simulink model "Prj2CDig_escalonado_gemeo_v2"  (R2026b)
settings: Solver=FixedStepDiscrete  StartTime=0  StopTime=StopTime  FixedStep=Ts
model workspace (MAT data in the model file):
  APlantCool = 0.758025026799
  APlantNom = [0.976809482048  0; 0  0.837999478908]
  BPlantCool = 0.0389974309185
  BPlantNom = [0.012391015895; 0.0114915598792]
  BetaCoolerSeno = 0.8
  CPlantCool = 0.00533973420046
  CPlantNom = [0.00104118199184 0.0230826408129]
  ConfirmacoesModo = 2
  FaseSeno = 2.9409972793
  KWVariavelParaPwm16 = 0
  Pwm16Max = 65535
  Pwm16Min = 0
  StopTime = 3600
  SubpassosGemeo = 6
  TaSim = 26.6
  Ts = 5.715
  TsSobre2 = 2.8575
  TsSubGemeo = 0.9525
  WBaseCooler = 3211
  WEntrarCooler = 2000
  WSairCooler = 1000
  YInicialGemeo = 27
  YInicialSim = 50
  cooler.y0 = 50
  cooler.u0 = 29668.6850394
  cooler.Nb = 2157.30127859
  cooler.Ki = 74.6363818008
  cooler.Kx = 9.0523214643
  cooler.Kq = 0.368257902254
  cooler.C = 0.00533973420046
  cooler.Cs = [1.21494479074 5.41983902077]
  cooler.Aod = [0.758025026799  0.0389974309185  0; 0  0.846686888484  5.41983902077; 0  -0.052237956106  0.846686888484]
  cooler.Bod = [0.0389974309185; 0; 0]
  cooler.Ld = [59.9192070008; -1100.25874176; -100.465858002]
  cooler.AdPlanta = 0.758025026799
  cooler.BdPlanta = 0.0389974309185
  cooler.CdPlanta = 0.00533973420046
  nominal.y0 = 50.50283
  nominal.u0 = 9688.13559322
  nominal.Nb = 1615.01542842
  nominal.Ki = 55.87486056
  nominal.Kx = [2.42292827 37.30035107]
  nominal.Kq = 0.45467056
  nominal.Cs = [1.30135744 5.41983902]
  nominal.GTermicoPwm16 = 455.85236927
  nominal.AdPlanta = [0.976809482048  0; 0  0.837999478908]
  nominal.BdPlanta = [0.012391015895; 0.0114915598792]
  nominal.CdPlanta = [0.00104118199184 0.0230826408129]
  nominal.Aod = [0.871488506271  -2.3349292179  0.012391015895  0; -0.0214603685254  0.362230610194  0.0114915598792  0; 0.547000658391  12.1268133919  0.846686888484  5.41983902077; 0.0988681165312  2.19187158404  -0.052237956106  0.846686888484]
  nominal.Bod = [0.012391015895; 0.0114915598792; 0; 0]
  nominal.Ld = [101.15520303; 20.6115440851; -525.365078033; -94.9575744738]
  nominal.Cod = [0.00104118199184 0.0230826408129 0 0]
  thetaGemeo = [0.00594308095276 0.00147339059286 0.0179875985617 0.0289186352165 1.00003134628e-05 0.0158089923599 4.45570940962e-05]
  vCenario = [5.715 26.6 3211 0.8 2.9409972793]
  vCool = [2.8575 50 29668.6850394 2157.30127859 74.6363818008 9.0523214643 0.368257902254 0.00533973420046 1.21494479074 5.41983902077]
  vNom = [2.8575 50.50283 9688.13559322 1615.01542842 55.87486056 2.42292827 37.30035107 0.45467056 1.30135744 5.41983902 455.85236927 0.976809482048 0.837999478908 0.012391015895 0.0114915598792]
  vPlanta = [50 50.50283 9688.13559322 50 29668.6850394 3211 0]
  vSupervisor = [2000 1000 2]
settings Model: Creator=Santana  LastModifiedBy=Santana

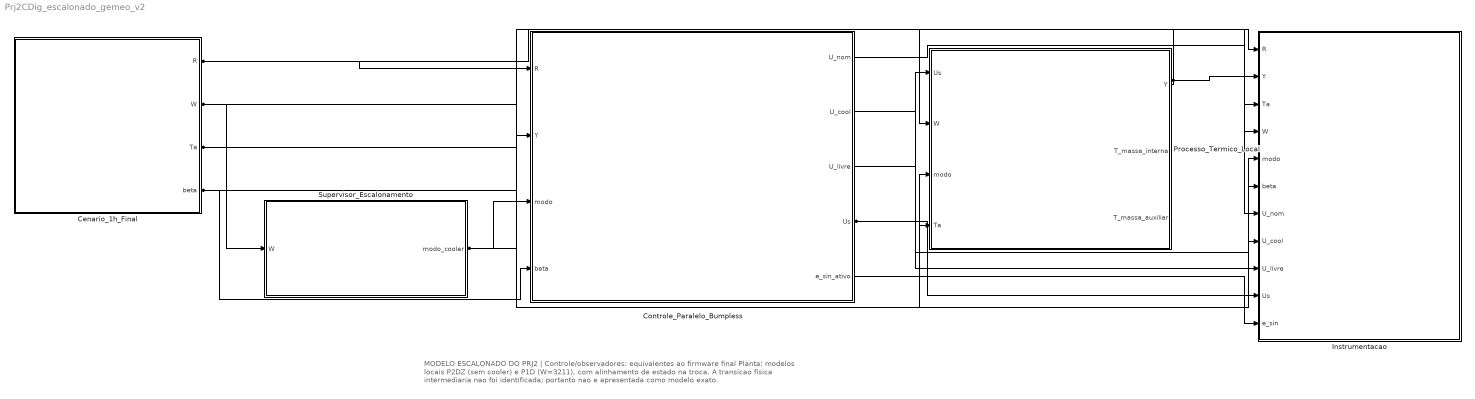
== system Prj2CDig_escalonado_gemeo_v2 ==
  note: MODELO ESCALONADO DO PRJ2  |  Controle/observadores: equivalentes ao firmware final
      | Planta: modelos locais P2DZ (sem cooler) e P1D (W=3211), com alinhamento de estado na troca.
      | A transicao fisica intermediaria nao foi identificada; portanto nao e apresentada como modelo exato.
  Cenario_1h_Final : Subsystem
  Controle_Paralelo_Bumpless : Subsystem
  Instrumentacao : Subsystem
  Processo_Termico_Local : Subsystem
  Supervisor_Escalonamento : Subsystem
  wires:
  Cenario_1h_Final/1(R) -> Controle_Paralelo_Bumpless/1(R), Instrumentacao/1(R)
  Cenario_1h_Final/2(W) -> Supervisor_Escalonamento/1(W), Processo_Termico_Local/2(W), Instrumentacao/4(W)
  Cenario_1h_Final/4(beta) -> Controle_Paralelo_Bumpless/4(beta), Instrumentacao/6(beta)
  Supervisor_Escalonamento/1(modo_cooler) -> Controle_Paralelo_Bumpless/3(modo), Processo_Termico_Local/3(modo), Instrumentacao/5(modo)
  Controle_Paralelo_Bumpless/4(Us) -> Processo_Termico_Local/1(Us), Instrumentacao/10(Us)
  Processo_Termico_Local/1(Y) -> Controle_Paralelo_Bumpless/2(Y), Instrumentacao/2(Y)
  Cenario_1h_Final/3(Ta) -> Instrumentacao/3(Ta), Processo_Termico_Local/4(Ta)
  Controle_Paralelo_Bumpless/1(U_nom) -> Instrumentacao/7(U_nom)
  Controle_Paralelo_Bumpless/2(U_cool) -> Instrumentacao/8(U_cool)
  Controle_Paralelo_Bumpless/3(U_livre) -> Instrumentacao/9(U_livre)
  Controle_Paralelo_Bumpless/5(e_sin_ativo) -> Instrumentacao/11(e_sin)

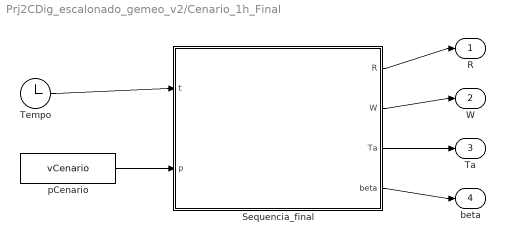
== system Prj2CDig_escalonado_gemeo_v2/Cenario_1h_Final ==
  Sequencia_final : MATLAB Function  TreatAsAtomicUnit=on
  Tempo : Clock
  pCenario : Constant  Value=vCenario
  R : Outport
  W : Outport  Port=2
  Ta : Outport  Port=3
  beta : Outport  Port=4
  wires:
  Tempo/1 -> Sequencia_final/1(t)
  pCenario/1 -> Sequencia_final/2(p)
  Sequencia_final/1(R) -> R/1
  Sequencia_final/2(W) -> W/1
  Sequencia_final/3(Ta) -> Ta/1
  Sequencia_final/4(beta) -> beta/1

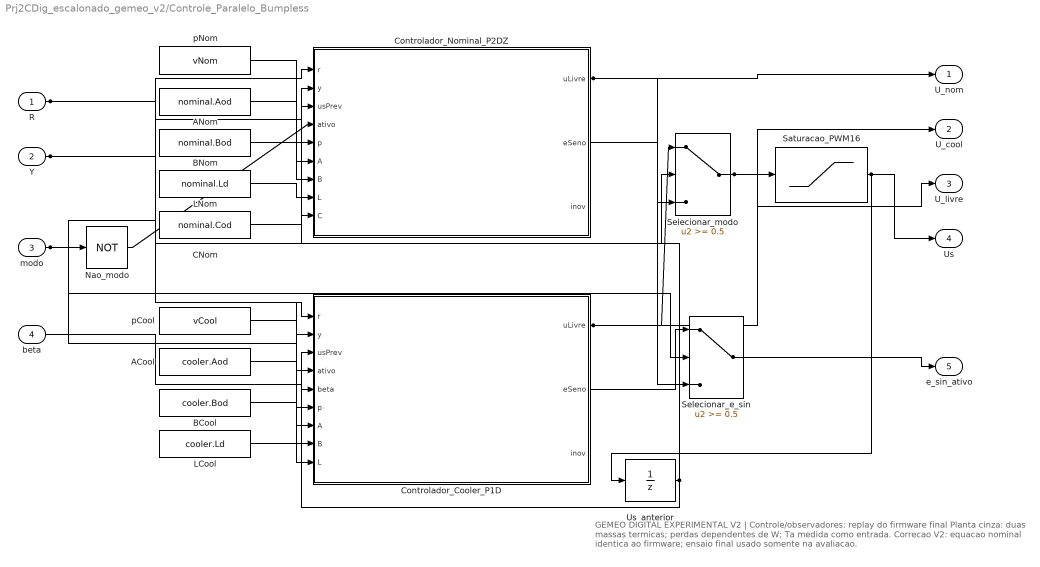
== system Prj2CDig_escalonado_gemeo_v2/Controle_Paralelo_Bumpless ==
  note: GEMEO DIGITAL EXPERIMENTAL V2  |  Controle/observadores: replay do firmware final
      | Planta cinza: duas massas termicas; perdas dependentes de W; Ta medida como entrada.
      | Correcao V2: equacao nominal identica ao firmware; ensaio final usado somente na avaliacao.
  R : Inport
  Y : Inport  Port=2
  modo : Inport  Port=3
  beta : Inport  Port=4
  ACool : Constant  Value=cooler.Aod
  ANom : Constant  Value=nominal.Aod
  BCool : Constant  Value=cooler.Bod
  BNom : Constant  Value=nominal.Bod
  CNom : Constant  Value=nominal.Cod
  Controlador_Cooler_P1D : MATLAB Function  TreatAsAtomicUnit=on
  Controlador_Nominal_P2DZ : MATLAB Function  TreatAsAtomicUnit=on
  LCool : Constant  Value=cooler.Ld
  LNom : Constant  Value=nominal.Ld
  Nao_modo : Logic  Operator=NOT  AllPortsSameDT=off  OutDataTypeStr=boolean
  Saturacao_PWM16 : Saturate  UpperLimit=Pwm16Max  LowerLimit=Pwm16Min
  Selecionar_e_sin : Switch  Threshold=0.5  SaturateOnIntegerOverflow=off  InputSameDT=off
  Selecionar_modo : Switch  Threshold=0.5  SaturateOnIntegerOverflow=off  InputSameDT=off
  Us_anterior : UnitDelay  SampleTime=Ts
  pCool : Constant  Value=vCool
  pNom : Constant  Value=vNom
  U_nom : Outport
  U_cool : Outport  Port=2
  U_livre : Outport  Port=3
  Us : Outport  Port=4
  e_sin_ativo : Outport  Port=5
  wires:
  R/1 -> Controlador_Nominal_P2DZ/1(r), Controlador_Cooler_P1D/1(r)
  Y/1 -> Controlador_Nominal_P2DZ/2(y), Controlador_Cooler_P1D/2(y)
  Us_anterior/1 -> Controlador_Nominal_P2DZ/3(usPrev), Controlador_Cooler_P1D/3(usPrev)
  modo/1 -> Nao_modo/1, Controlador_Cooler_P1D/4(ativo), Selecionar_modo/2, Selecionar_e_sin/2
  Nao_modo/1 -> Controlador_Nominal_P2DZ/4(ativo)
  beta/1 -> Controlador_Cooler_P1D/5(beta)
  pNom/1 -> Controlador_Nominal_P2DZ/5(p)
  ANom/1 -> Controlador_Nominal_P2DZ/6(A)
  BNom/1 -> Controlador_Nominal_P2DZ/7(B)
  LNom/1 -> Controlador_Nominal_P2DZ/8(L)
  CNom/1 -> Controlador_Nominal_P2DZ/9(C)
  pCool/1 -> Controlador_Cooler_P1D/6(p)
  ACool/1 -> Controlador_Cooler_P1D/7(A)
  BCool/1 -> Controlador_Cooler_P1D/8(B)
  LCool/1 -> Controlador_Cooler_P1D/9(L)
  Controlador_Cooler_P1D/1(uLivre) -> Selecionar_modo/1, U_cool/1
  Controlador_Nominal_P2DZ/1(uLivre) -> Selecionar_modo/3, U_nom/1
  Selecionar_modo/1 -> Saturacao_PWM16/1, U_livre/1
  Saturacao_PWM16/1 -> Us_anterior/1, Us/1
  Controlador_Cooler_P1D/2(eSeno) -> Selecionar_e_sin/1
  Controlador_Nominal_P2DZ/2(eSeno) -> Selecionar_e_sin/3
  Selecionar_e_sin/1 -> e_sin_ativo/1

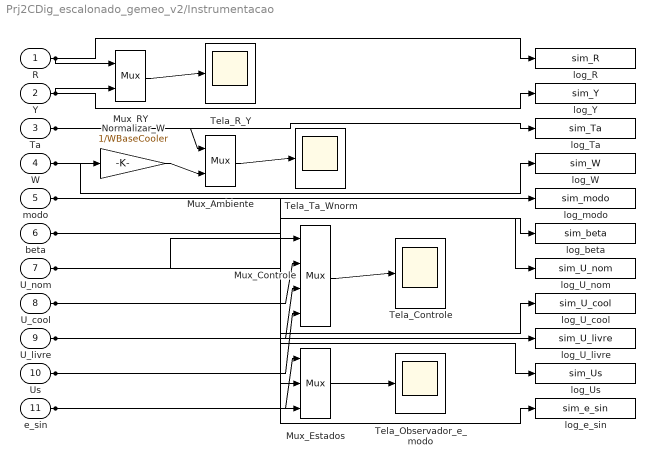
== system Prj2CDig_escalonado_gemeo_v2/Instrumentacao ==
  R : Inport
  Y : Inport  Port=2
  Ta : Inport  Port=3
  W : Inport  Port=4
  modo : Inport  Port=5
  beta : Inport  Port=6
  U_nom : Inport  Port=7
  U_cool : Inport  Port=8
  U_livre : Inport  Port=9
  Us : Inport  Port=10
  e_sin : Inport  Port=11
  Mux_Ambiente : Mux  Inputs=2
  Mux_Controle : Mux
  Mux_Estados : Mux  Inputs=3
  Mux_RY : Mux  Inputs=2
  Normalizar_W : Gain  Gain=1/WBaseCooler
  Tela_Controle : Scope
  Tela_Observador_e_modo : Scope
  Tela_R_Y : Scope
  Tela_Ta_Wnorm : Scope
  log_R : ToWorkspace  VariableName=sim_R  SaveFormat=Timeseries  SampleTime=-1
  log_Ta : ToWorkspace  VariableName=sim_Ta  SaveFormat=Timeseries  SampleTime=-1
  log_U_cool : ToWorkspace  VariableName=sim_U_cool  SaveFormat=Timeseries  SampleTime=-1
  log_U_livre : ToWorkspace  VariableName=sim_U_livre  SaveFormat=Timeseries  SampleTime=-1
  log_U_nom : ToWorkspace  VariableName=sim_U_nom  SaveFormat=Timeseries  SampleTime=-1
  log_Us : ToWorkspace  VariableName=sim_Us  SaveFormat=Timeseries  SampleTime=-1
  log_W : ToWorkspace  VariableName=sim_W  SaveFormat=Timeseries  SampleTime=-1
  log_Y : ToWorkspace  VariableName=sim_Y  SaveFormat=Timeseries  SampleTime=-1
  log_beta : ToWorkspace  VariableName=sim_beta  SaveFormat=Timeseries  SampleTime=-1
  log_e_sin : ToWorkspace  VariableName=sim_e_sin  SaveFormat=Timeseries  SampleTime=-1
  log_modo : ToWorkspace  VariableName=sim_modo  SaveFormat=Timeseries  SampleTime=-1
  wires:
  Mux_RY/1 -> Tela_R_Y/1
  R/1 -> Mux_RY/1, log_R/1
  Y/1 -> Mux_RY/2, log_Y/1
  Mux_Ambiente/1 -> Tela_Ta_Wnorm/1
  Ta/1 -> Mux_Ambiente/1, log_Ta/1
  W/1 -> Normalizar_W/1, log_W/1
  Normalizar_W/1 -> Mux_Ambiente/2
  Mux_Controle/1 -> Tela_Controle/1
  U_nom/1 -> Mux_Controle/1, log_U_nom/1
  U_cool/1 -> Mux_Controle/2, log_U_cool/1
  U_livre/1 -> Mux_Controle/3, log_U_livre/1
  Us/1 -> Mux_Controle/4, log_Us/1
  Mux_Estados/1 -> Tela_Observador_e_modo/1
  e_sin/1 -> Mux_Estados/1, log_e_sin/1
  modo/1 -> Mux_Estados/2, log_modo/1
  beta/1 -> Mux_Estados/3, log_beta/1

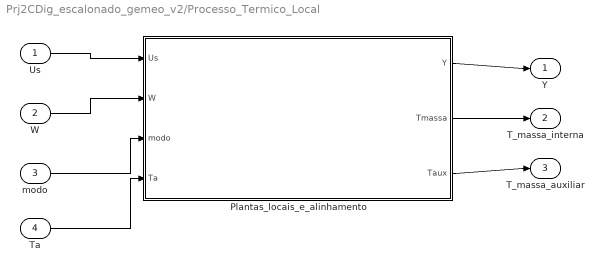
== system Prj2CDig_escalonado_gemeo_v2/Processo_Termico_Local ==
  Us : Inport
  W : Inport  Port=2
  modo : Inport  Port=3
  Ta : Inport  Port=4
  Plantas_locais_e_alinhamento : MATLAB Function  TreatAsAtomicUnit=on
  Y : Outport
  T_massa_interna : Outport  Port=2
  T_massa_auxiliar : Outport  Port=3
  wires:
  Us/1 -> Plantas_locais_e_alinhamento/1(Us)
  W/1 -> Plantas_locais_e_alinhamento/2(W)
  modo/1 -> Plantas_locais_e_alinhamento/3(modo)
  Plantas_locais_e_alinhamento/1(Y) -> Y/1
  Plantas_locais_e_alinhamento/2(Tmassa) -> T_massa_interna/1
  Plantas_locais_e_alinhamento/3(Taux) -> T_massa_auxiliar/1
  Ta/1 -> Plantas_locais_e_alinhamento/4(Ta)

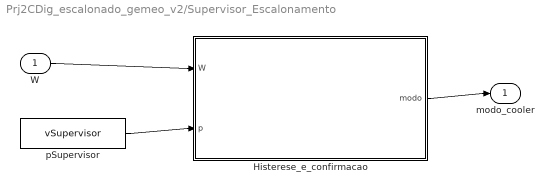
== system Prj2CDig_escalonado_gemeo_v2/Supervisor_Escalonamento ==
  W : Inport
  Histerese_e_confirmacao : MATLAB Function  TreatAsAtomicUnit=on
  pSupervisor : Constant  Value=vSupervisor
  modo_cooler : Outport
  wires:
  W/1 -> Histerese_e_confirmacao/1(W)
  pSupervisor/1 -> Histerese_e_confirmacao/2(p)
  Histerese_e_confirmacao/1(modo) -> modo_cooler/1

== matlab function Prj2CDig_escalonado_gemeo_v2/Supervisor_Escalonamento/Histerese_e_confirmacao ==
  data: W input size=1; modo output size=1; p input size=[1 3]
function modo = f(W,p)
%#codegen
persistent estado contador
if isempty(estado), estado=false; contador=uint8(0); end
if estado, pedido=(W>p(2)); else, pedido=(W>=p(1)); end
if pedido==estado
    contador=uint8(0);
else
    contador=contador+uint8(1);
    if contador>=uint8(p(3)), estado=pedido; contador=uint8(0); end
end
modo=double(estado);
end

== matlab function Prj2CDig_escalonado_gemeo_v2/Cenario_1h_Final/Sequencia_final ==
  data: t input size=1; R output size=1; p input size=[1 5]; W output size=1; Ta output size=1; beta output size=1
function [R,W,Ta,beta] = f(t,p)
%#codegen
Ts=p(1); Ta=p(2); Wbase=p(3); betaSeno=p(4); fase=p(5);
amostra=floor((t+1e-9)/Ts);
if mod(floor(amostra/70),2)==0, R=45; else, R=55; end
if t<1000
    W=0;
elseif t<1800 || t>=3000
    W=Wbase;
else
    W=3051+803*sin(2*pi*(t-1800)/64+fase);
    if t>=2936
        a=0.5*(1+cos(pi*(t-2936)/64));
        W=Wbase+a*(W-Wbase);
    end
    W=min(max(W,2248),3854);
end
if t>=1800 && t<3000, beta=betaSeno; else, beta=1; end
end

== matlab function Prj2CDig_escalonado_gemeo_v2/Controle_Paralelo_Bumpless/Controlador_Nominal_P2DZ ==
  data: r input size=1; uLivre output size=1; y input size=1; usPrev input size=1; ativo input size=1; p input size=[1 15]; A input size=[4 4]; B input size=[4 1]; L input size=[4 1]; C input size=[1 4]; eSeno output size=1; inov output size=1
function [uLivre,eSeno,inov] = f(r,y,usPrev,ativo,p,A,B,L,C)
%#codegen
persistent z xi eAnt rAnt corrAnt q inovAnt uAnt yGuard rGuard ativoAnt iniciado
Ts2=p(1); y0=p(2); u0=p(3); Nb=p(4); Ki=p(5);
K1=p(6); K2=p(7); Kq=p(8); Cs1=p(9); Cs2=p(10);
G=p(11); ad1=p(12); ad2=p(13); bd1=p(14); bd2=p(15);
uLivre=0.0; eSeno=0.0; inov=0.0;
if isempty(iniciado)
    entradaEq=(y-y0)*G;
    z=[bd1*entradaEq/(1-ad1);bd2*entradaEq/(1-ad2);0;0];
    q=usPrev-u0; xi=(usPrev-u0-Nb*(r-y0)+K1*z(1)+K2*z(2)+Kq*q)/Ki;
    eAnt=r-y; rAnt=r; corrAnt=0; inovAnt=0; uAnt=usPrev;
    yGuard=y; rGuard=r; ativoAnt=false; iniciado=true;
else
    if ativoAnt
        z=A*z+B*q+L*(yGuard-y0); q=usPrev-u0; corrAnt=(usPrev-uAnt)/Ki;
    else
        entradaEq=(yGuard-y0)*G;
        z=[bd1*entradaEq/(1-ad1);bd2*entradaEq/(1-ad2);0;0]; q=usPrev-u0;
        xi=(usPrev-u0-Nb*(rGuard-y0)+K1*z(1)+K2*z(2)+Kq*q)/Ki;
        eAnt=rGuard-yGuard; rAnt=rGuard; corrAnt=0;
    end
end
erro=r-y; xi=xi+Ts2*(eAnt+rAnt-y)+corrAnt;
eSeno=Cs1*z(3)+Cs2*z(4); inov=y-y0-C*z;
uLivre=u0+Nb*(r-y0)+Ki*xi-K1*z(1)-K2*z(2)-Kq*q-eSeno;
eAnt=erro; rAnt=r; inovAnt=inov; uAnt=uLivre;
yGuard=y; rGuard=r; ativoAnt=(ativo>=0.5);
end

== matlab function Prj2CDig_escalonado_gemeo_v2/Controle_Paralelo_Bumpless/Controlador_Cooler_P1D ==
  data: r input size=1; uLivre output size=1; y input size=1; usPrev input size=1; ativo input size=1; beta input size=1; p input size=[1 10]; A input size=[3 3]; B input size=[3 1]; L input size=[3 1]; eSeno output size=1; inov output size=1
function [uLivre,eSeno,inov] = f(r,y,usPrev,ativo,beta,p,A,B,L)
%#codegen
persistent z xi eAnt rAnt corrAnt q inovAnt uAnt yGuard rGuard ativoAnt betaAnt iniciado
Ts2=p(1); y0=p(2); u0=p(3); Nb=p(4); Ki=p(5);
Kx=p(6); Kq=p(7); Cp=p(8); Cs1=p(9); Cs2=p(10);
uLivre=0.0; eSeno=0.0; inov=0.0;
if isempty(iniciado)
    z=[(y-y0)/Cp;0;0]; q=usPrev-u0; betaAnt=beta;
    xi=(usPrev-u0-Nb*beta*(r-y0)+Kx*z(1)+Kq*q)/Ki;
    eAnt=r-y; rAnt=r; corrAnt=0; inovAnt=0; uAnt=usPrev;
    yGuard=y; rGuard=r; ativoAnt=false; iniciado=true;
else
    if ativoAnt
        z=A*z+B*q+L*inovAnt; q=usPrev-u0; corrAnt=(usPrev-uAnt)/Ki;
    else
        z=[(yGuard-y0)/Cp;0;0]; q=usPrev-u0;
        xi=(usPrev-u0-Nb*betaAnt*(rGuard-y0)+Kx*z(1)+Kq*q)/Ki;
        eAnt=rGuard-yGuard; rAnt=rGuard; corrAnt=0;
    end
end
if abs(beta-betaAnt)>1e-12
    xi=xi+Nb*(betaAnt-beta)*(r-y0)/Ki; betaAnt=beta;
end
erro=r-y; xi=xi+Ts2*(eAnt+rAnt-y)+corrAnt;
eSeno=Cs1*z(2)+Cs2*z(3); inov=y-y0-Cp*z(1);
uLivre=u0+Nb*beta*(r-y0)+Ki*xi-Kx*z(1)-Kq*q-eSeno;
eAnt=erro; rAnt=r; inovAnt=inov; uAnt=uLivre;
yGuard=y; rGuard=r; ativoAnt=(ativo>=0.5);
end

== matlab function Prj2CDig_escalonado_gemeo_v2/Processo_Termico_Local/Plantas_locais_e_alinhamento ==
  data: Us input size=1; Y output size=1; W input size=1; modo input size=1; Tmassa output size=1; Taux output size=1; Ta input size=1; thetaGemeo parameter size=[1 7]; TsSubGemeo parameter size=1; SubpassosGemeo parameter size=1; YInicialGemeo parameter size=1
function [Y,Tmassa,Taux] = f(Us,W,modo,Ta, thetaGemeo, TsSubGemeo, SubpassosGemeo, YInicialGemeo)
%#codegen
persistent x uAtrasado iniciado
if isempty(iniciado)
    x=zeros(2,1); uAtrasado=0; iniciado=true;
end
th=thetaGemeo;
a12=th(1); a21=th(2); a10=th(3);
a1w=th(4); a20=th(5); a2w=th(6); bU=th(7);
Tabs=x+[YInicialGemeo;YInicialGemeo];
Y=Tabs(1); Tmassa=Tabs(2); Taux=Tabs(2); Wnorm=min(max(W/3211,0),1.25);
a1=a10+a1w*Wnorm; a2=a20+a2w*Wnorm;
for j=1:SubpassosGemeo
    dx1=-(a12+a1)*Tabs(1)+a12*Tabs(2)+bU*uAtrasado+a1*Ta;
    dx2=a21*Tabs(1)-(a21+a2)*Tabs(2)+a2*Ta;
    Tabs=Tabs+TsSubGemeo*[dx1;dx2];
end
x=Tabs-[YInicialGemeo;YInicialGemeo];
uAtrasado=Us;
end
